simulink model "ModelLLCController"  (R2026a)
settings: Solver=ode23t  StopTime=5e-3  FixedStep=1e-4  MaxStep=1/(10*llcCompensator.resonantFrequency)  AbsTol=1e-3
PreLoadFcn:
  | % Parameterize the model
  | 
  | if ~exist('LLCDesign', 'var')
  | LLCConverterDefaultInputParameters;
  | end
undefined symbols (not defined in the file or in its folder): llcCompensator, LLCController
libraries: fl_lib x52, nesl_utility x34, ee_lib x27, ConverterLibrary x1
(part 1 of 4)
Description:
  | Design of LLC Resonant Converter
settings Model: SimulationMode=accelerator  ExtModeTrigDuration=100  Creator=The MathWorks, Inc.  LastModifiedBy=vsolaise
settings SolverCC: MaxConsecutiveMinStep=10
settings DataIOCC: StateSaveName=tmp_raccel_xout  SignalLoggingName=logsoutLLCConverter  OutputTimes=[0:1.1*3*Voc/(1*2000):1.1*3*Voc/1]
settings OptimizationCC: EfficientMapNaN2IntZero=off
settings HardwareCC: ProdHWDeviceType=Intel->x86-32 (Windows32)  TargetBitPerPointer=64.0  TargetBitPerSizeT=64.0  TargetBitPerPtrDiffT=64.0  TargetLongLongMode=on  TargetIntDivRoundTo=Zero  TargetEndianess=LittleEndian  TargetWordSize=64.0  TargetHWDeviceType=MATLAB Host  ProdEqTarget=off
settings RTWCC: SystemTargetFile=raccel.tlc  TemplateMakefile=raccel_default_tmf  RTWVerbose=off  RTWUseSimCustomCode=on
settings CodeAppCC: GenerateComments=off  MaxIdLength=128.0  SimulinkBlockComments=off
settings RaccelTargetCC: ExtModeTransport=0.0  ExtModeStaticAllocSize=1000000.0  ENABLE_SLEXEC_SSBRIDGE=1.0  RTWCAPIParams=on  RTWCAPIRootIO=on  MultiwordLength=2048.0
settings SimscapeCC: SimscapeNominalValues="[{\"value\":\"1\",\"unit\":\"A\"},{\"value\":\"1\",\"unit\":\"bar\"},{\"value\":\"1\",\"unit\":\"cm^2\"},{\"value\":\"1\",\"unit\":\"cm^3/s\"},{\"value\":\"1\",\"unit\":\"kJ/kg\"},{\"value\":\"1\",\"unit\":\"kW\"},{\"value\":\"1\",\"unit\":\"l\"},{\"value\":\"1\",\"unit\":\"N\"},{\"value\":\"1\",\"unit\":\"N*m\"},{\"value\":\"1\",\"unit\":\"V\"}]"  SimscapeLogName=SimlogLLCConverter  SimscapeLogLimitData=off  SimscapeLogDataHistory=5000.0

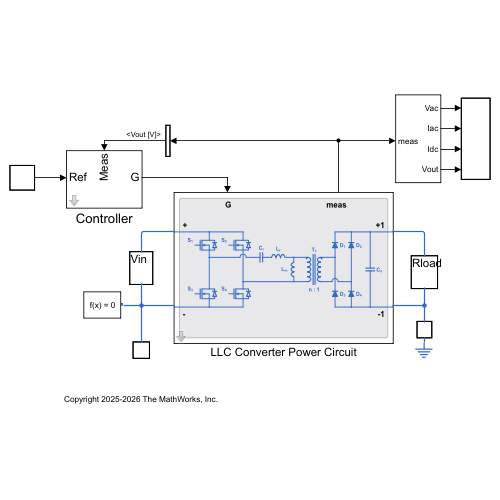
[thumbnail: Simulink's stored preview of the top-level diagram]
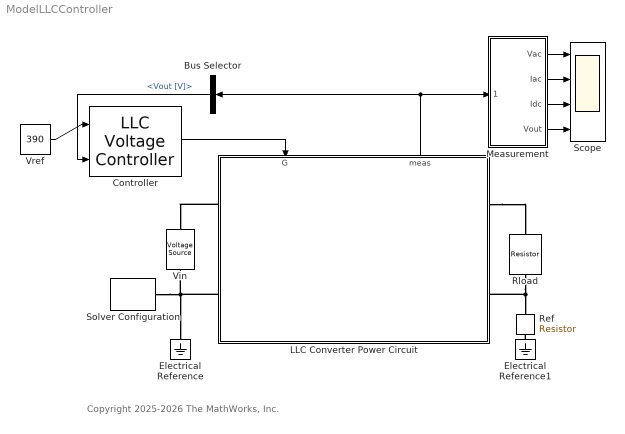
== system ModelLLCController ==
  note: Copyright 2025-2026 The MathWorks, Inc.
  Bus Selector : BusSelector  OutputSignals=Rectifier.Vout [V]
  Controller : ConverterLibrary/Controller/Soft-Switching Converters/LLC Voltage Controller  resFreq=llcCompensator.resonantFrequency  Fmin=llcCompensator.minPUfrequency  Fmax=llcCompensator.maxPUfrequency  Tdead=llcCompensator.deadTime  cntrlSelect=PI controller (Continuous)  VdcValue=LLCSpec.maxInputVoltage.value  Kc=llcCompensator.Ki  numSdomain=llcCompensator.numSDomain  denSdomain=llcCompensator.denSDomain  numZdomain=llcCompensator.numZDomain  denZdomain=llcCompensator.denZDomain  Kp=LLCController.Kp  Ki=LLCController.Ki  TsController=LLCController.Ts  vcoSelect=Two rate  vcoGain=llcCompensator.constantVCOGain  vcoGainVec=llcCompensator.constantVCOGain*[1 1]  pwmSampleTime=1e-7
      link override 2P2Z Compensator: LabelModeActiveChoice=PIContinuous
      link override VCO: LabelModeActiveChoice=TwoRate
      settings: SourceProductName=Simscape Power Converter Components
  Electrical Reference : fl_lib/Electrical/Electrical Elements/Electrical Reference
  Electrical Reference1 : fl_lib/Electrical/Electrical Elements/Electrical Reference
  LLC Converter Power Circuit : Subsystem  mask(LLC Converter Plant){llcConverterModel=Detailed Full-Bridge, ratedPower=10e3, ratedPower_unit=W, VIn=380, VIn_unit=V, Cr=3.3703e-7, Cr_unit=F, seriesInductorOption=Use transformer leakage inductance, Lr=30, Lr_unit=uH, RLr=0, RLr_unit=mOhm, Llk1=7.14e-6, Llk1_unit=H, R1=0.01, R1_unit=Ohm, Llk2=4.0645e-7, Llk2_unit=H, R2=0.01, R2_unit=Ohm, Lm=9.7705e-5, Lm_unit=H, n=0.96154, Cf=7.1111e-4, Cf_unit=F, Esr=0.02, Esr_unit=Ohm, Vco=350, Vco_unit=V, primaryDeviceOption=Ideal Semiconductor Switch, RdsOn=0.001, RdsOn_unit=Ohm, GdsOff=1e-5, GdsOff_unit=1/Ohm, Vth=2.5, Vth_unit=V, VfBody=0.6, VfBody_unit=V, RdBody=0.001, RdBody_unit=Ohm, GdBody=1e-5, GdBody_unit=1/Ohm, Cdsparasitic=2e-10, Cdsparasitic_unit=F, simTempPri=25, simTempPri_unit=degC, rectifierOption=Full Bridge, secondaryDeviceOption=Ideal Diode, VfSec=0.6, VfSec_unit=V, RdSec=0.001, RdSec_unit=Ohm, GdSec=1e-5, GdSec_unit=1/Ohm, simTempSec=25, simTempSec_unit=degC}
      mask prompts: llcConverterModel "LLC Converter model"; ratedPower "Rated power (P)"; VIn "Nominal input voltage (Vdc)"; Cr "Resonant capacitance (Cr)"; seriesInductorOption "Series resonant inductance"; Lr "Series resonant inductance (Lr)"; RLr "Series inductance resistance"; Llk1 "Primary leakage inductance (Lr)"; R1 "Primary resistance (R1)"; Llk2 "Secondary leakage inductance (Llk2)"; R2 "Secondary resistance (R2)"; Lm "Magnetizing inductance (Lm)"; n "Transformer turns ratio (n)"; Cf "Output filter capacitance (Co)"; Esr "Output filter capacitor ESR (Rco)"; Vco "Initial output capacitor voltage"; primaryDeviceOption "Select the primary switching device"; RdsOn "On-state resistance"; GdsOff "Off-state conductance"; Vth "Threshold voltage"; VfBody "Body diode forward voltage"; RdBody "Body diode on-resistance"; GdBody "Body diode off-conductance"; Cdsparasitic "MOSFET parasitic capacitance"; simTempPri "Simulation temperature"; rectifierOption "Select the rectifier topology"; secondaryDeviceOption "Select the secondary diode"; VfSec "Forward voltage"; RdSec "On resistance"; GdSec "Off conductance"; simTempSec "Simulation temperature"
      mask help: This block models the power circuit of the LLC resonant converter. You can choose between different switch and diode models. For the primary semiconductor switch, you can choose between ideal semiconductor switch, MOSFET without thermal port and tabulated MOSFET with thermal port. For the secondary, you can choose between ideal and tabulated diode.
      mask init:
      | %% Unit conversion: convert displayed values to base SI units
      | convMap = containers.Map( ...
      |     {'W','kW','MW','V','kV','mV','F','mF','uF','nF','pF', ...
      |      'H','mH','uH','nH','Ohm','kOhm','mOhm','S','mS','1/Ohm'}, ...
      |     {1, 1e3, 1e6, 1, 1e3, 1e-3, 1, 1e-3, 1e-6, 1e-9, 1e-12, ...
      |      1, 1e-3, 1e-6, 1e-9, 1, 1e3, 1e-3, 1, 1e-3, 1});
      | ratedPower = ratedPower * convMap(ratedPower_unit);
      | VIn = VIn * convMap(VIn_unit);
      | Cr = Cr * convMap(Cr_unit);
      | Lr_SI = Lr * convMap(Lr_unit);
      | RLr_SI = RLr * convMap(RLr_unit);
      | Llk1 = Llk1 * convMap(Llk1_unit);
      | R1 = R1 * convMap(R1_unit);
      | Llk2 = Llk2 * convMap(Llk2_unit);
      | R2 = R2 * convMap(R2_unit);
      | Lm = Lm * convMap(Lm_unit);
      | Cf = Cf * convMap(Cf_unit);
      | Esr = Esr * convMap(Esr_unit);
      | Vco_SI = Vco * convMap(Vco_unit);
      | RdsOn = RdsOn * convMap(RdsOn_unit);
      | GdsOff = GdsOff * convMap(GdsOff_unit);
      | Vth = Vth * convMap(Vth_unit);
      | VfBody = VfBody * convMap(VfBody_unit);
      | RdBody = RdBody * convMap(RdBody_unit);
      | GdBody = GdBody * convMap(GdBody_unit);
      | Cdsparasitic = Cdsparasitic * convMap(Cdsparasitic_unit);
      | VfSec = VfSec * convMap(VfSec_unit);
      | RdSec = RdSec * convMap(RdSec_unit);
      | GdSec = GdSec * convMap(GdSec_unit);
      | %% Transformer turns ratio and leakage inductances
      | % A centre-tap rectifier halves the ratio and doubles the secondary leakage of the
      | % centre-tapped transformer. With an external series inductor the leakages are a small
      | % share of it, referred to each winding, so they are never zero.
      | leakageShareOfExternalInductor = 1e-3;
      | primaryLeakage = Llk1;
      | secondaryLeakage = Llk2;
      | % Read by name: seriesInductorOption is an evaluated popup, so its workspace value is an index
      | if strcmp(get_param(gcb, 'seriesInductorOption'), 'Use external inductance') && startsWith(get_param(gcb, 'llcConverterModel'), 'Detailed')
      |     primaryLeakage = leakageShareOfExternalInductor*Lr_SI;
      |     secondaryLeakage = leakageShareOfExternalInductor*Lr_SI/n^2;
      | end
      | if ~(isfinite(primaryLeakage) && primaryLeakage > 0 && isfinite(secondaryLeakage) && secondaryLeakage > 0)
      |     error('The transformer leakage inductances must be positive. Primary: %g H, secondary: %g H.', ...
      |         primaryLeakage, secondaryLeakage);
      | end
      | if strcmp(rectifierOption, 'Centre-Tap')
      |     xfmrTurnsRatio = n/2;
      |     xfmrSecondaryLeakage = 2*secondaryLeakage;
      | else
      |     xfmrTurnsRatio = n;
      |     xfmrSecondaryLeakage = secondaryLeakage;
      | end
      | xfmrPrimaryLeakage = primaryLeakage;
      | %% Simulation temperature (loss-only, thermal MOSFET device)
      | % Temperature is an OFFSET unit (K = degC + 273.15), so it cannot use the
      | % multiplicative convMap above; convert it explicitly. simTempPri_K is read
      | % directly by each thermal MOSFET's junction-temperature initial target and by
      | % each Temperature Source in the primary bridge.
      | if strcmp(simTempPri_unit, 'degC')
      |     simTempPri_K = simTempPri + 273.15;
      | elseif strcmp(simTempPri_unit, 'K')
      |     simTempPri_K = simTempPri;
      | else
      |     error('LLC Converter Power Circuit: unrecognized simulation-temperature unit "%s" (expected degC or K).', simTempPri_unit);
      | end
      | %% Simulation temperature (secondary rectifier, tabulated diode)
      | % Same offset-unit conversion as the primary above (K = degC + 273.15), which is why
      | % neither can use the multiplicative convMap. simTempSec_K is read by every tabulated
      | % rectifier diode's device simulation temperature. That is the only temperature input
      | % those blocks have: in this configuration the diode has two electrical ports and no
      | % thermal port, so a junction-temperature target on it would be inert.
      | if strcmp(simTempSec_unit, 'degC')
      |     simTempSec_K = simTempSec + 273.15;
      | elseif strcmp(simTempSec_unit, 'K')
      |     simTempSec_K = simTempSec;
      | else
      |     error('LLC Converter Power Circuit: unrecognized simulation-temperature unit "%s" (expected degC or K).', simTempSec_unit);
      | end
      | %% Select model variant and visibility
      | selectLLCPlantModel(gcb);
      | %% Block icon
      | % The icon is drawn by the mask Display code, which resolves its four artwork files
      | % (FullBridgeLLCCentreTapRectifier.svg and siblings) by name from the MATLAB path.
      | % They live in Components/ConverterPlants/CombinedLLCConverterPlant/icons, which
      | % the project puts on the path. An earlier design kept the SVG source in
      | % model-workspace variables and unpacked it to tempdir here; those variables no longer
      | % exist, so that code only stranded a file handle on a zero-byte temp file every run.
      settings: CopyFcn="set_param(gcbh,\"LinkStatus\",\"none\");"  PortSchema="{\"entries\":[{\"content\":{\"sides\":[{\"content\":{\"connectorIds\":[\"LConn1\",\"LConn2\"]},\"type\":\"ConnectorPlacement.EquallySpacedRectSide\",\"uuid\":\"7d0af355-cbc1-43de-86a8-478c0417a0e6\"},{\"content\":{\"connectorIds\":[\"RConn1\",\"RConn2\"],\"side\":\"RIGHT\"},\"type\":\"ConnectorPlacement.EquallySpacedRectSide\",\"uuid\":\"e5e2e9fd-b3a0-4f29-84de-d1d266c8101b\"},{\"content\":{\"connectorIds\":[\"In1\",\"Out1\"],\"side\":\"TOP\"},\"type\":\"ConnectorPlacement.EquallySpacedRectSide\",\"uuid\":\"2a0404a0-819d-4dd0-9f33-52ca4a6707b9\"}]},\"type\":\"ConnectorPlacement.EquallySpacedConnector\",\"uuid\":\"862cc0c4-78b7-4235-be37-b455f1ccafcc\"}],\"packageUris\":[\"http://schema.mathworks.com/mf0/Connector/R2020b\"],\"version\":\"1.0\"}"
      mask Help: web('LLCConverterPlant.html')
      mask TypeOptions llcConverterModel: Simplified Half-Bridge | Detailed Half-Bridge | Detailed Full-Bridge
      mask Callback llcConverterModel: selectLLCPlantModel(gcb);
      mask TypeOptions ratedPower_unit: W | kW | MW
      mask TypeOptions VIn_unit: V | kV | mV
      mask TypeOptions Cr_unit: F | mF | uF | nF | pF
      mask TypeOptions seriesInductorOption: Use external inductance | Use transformer leakage inductance
      mask Callback seriesInductorOption: selectLLCSeriesInductor(gcb);
      mask TypeOptions Lr_unit: H | mH | uH | nH
      mask TypeOptions RLr_unit: Ohm | mOhm | kOhm
      mask TypeOptions Llk1_unit: H | mH | uH | nH
      mask TypeOptions R1_unit: Ohm | kOhm | mOhm
      mask TypeOptions Llk2_unit: H | mH | uH | nH
      mask TypeOptions R2_unit: Ohm | kOhm | mOhm
      mask TypeOptions Lm_unit: H | mH | uH | nH
      mask TypeOptions Cf_unit: F | mF | uF | nF | pF
      mask TypeOptions Esr_unit: Ohm | kOhm | mOhm
      mask TypeOptions Vco_unit: V | kV | mV
      mask TypeOptions primaryDeviceOption: Ideal Semiconductor Switch | MOSFET (Ideal, Switching) with Thermal
      mask Callback primaryDeviceOption: selectLLCPlantPrimaryMOSFET(gcb);
      mask TypeOptions RdsOn_unit: Ohm | kOhm | mOhm
      mask TypeOptions GdsOff_unit: 1/Ohm | S | mS
      mask TypeOptions Vth_unit: V | kV | mV
      mask TypeOptions VfBody_unit: V | mV
      mask TypeOptions RdBody_unit: Ohm | kOhm | mOhm
      mask TypeOptions GdBody_unit: 1/Ohm | S | mS
      mask TypeOptions Cdsparasitic_unit: F | mF | uF | nF | pF
      mask TypeOptions simTempPri_unit: degC | K
      mask TypeOptions rectifierOption: Centre-Tap | Full Bridge
      mask Callback rectifierOption: selectLLCPlantSecondaryDiode(gcb);
      mask TypeOptions secondaryDeviceOption: Ideal Diode | Tabulated Diode
      mask Callback secondaryDeviceOption: selectLLCPlantSecondaryDiode(gcb);
      mask TypeOptions VfSec_unit: V | mV
      mask TypeOptions RdSec_unit: Ohm | kOhm | mOhm
      mask TypeOptions GdSec_unit: 1/Ohm | S | mS
      mask TypeOptions simTempSec_unit: degC | K
      mask DialogControl LLCTank Prompt: Resonant tank parameters
      mask DialogControl Switch Prompt: Primary Inverter
      mask DialogControl openMOSFETMask Prompt: Open the MOSFET block mask
      mask DialogControl openMOSFETMask Callback:
      | blockPath = [gcb, '/LLC Primary Inverter and Resonant Tank/LLC Detailed Model/Inverter/Primary Inverter'];
      | llcConverterChoice = get_param(gcb,'llcConverterModel');
      | switch llcConverterChoice
      |     case 'Detailed Half-Bridge'
      |         open_system([blockPath, '/Half Bridge with Thermal/MOSFETA1'], 'mask');
      |     case 'Detailed Full-Bridge'
      |         open_system([blockPath, '/Full Bridge with Thermal/MOSFETA1'], 'mask');
      |     otherwise
      |         error('Open the MOSFET mask only in a Detailed model with the thermal MOSFET device selected.');
      | end
      mask DialogControl applyMOSFETParam Prompt: Apply parameters to all primary MOSFET blocks
      mask DialogControl applyMOSFETParam Callback:
      | llcConverterChoice = get_param(gcb, 'llcConverterModel');
      | primaryInvBase = [gcb, '/LLC Primary Inverter and Resonant Tank/LLC Detailed Model/Inverter/Primary Inverter'];
      | switch llcConverterChoice
      |     case 'Detailed Half-Bridge'
      |         srcBlock = [primaryInvBase, '/Half Bridge with Thermal/MOSFETA1'];
      |         dstBlocks = {[primaryInvBase, '/Half Bridge with Thermal/MOSFETA2']};
      |     case 'Detailed Full-Bridge'
      |         srcBlock = [primaryInvBase, '/Full Bridge with Thermal/MOSFETA1'];
      |         dstBlocks = {[primaryInvBase, '/Full Bridge with Thermal/MOSFETA2'], [primaryInvBase, '/Full Bridge with Thermal/MOSFETB1'], [primaryInvBase, '/Full Bridge with Thermal/MOSFETB2']};
      |     otherwise
      |         return;
      | end
      | paramNames = fieldnames(get_param(srcBlock, 'DialogParameters'));
      | paramValues = cellfun(@(x) get_param(srcBlock, x), paramNames, 'UniformOutput', false);
      | for k = 1:numel(dstBlocks)
      |     cellfun(@(x, y) set_param(dstBlocks{k}, x, y), paramNames, paramValues, 'UniformOutput', false);
      | end
      | fprintf('Applied MOSFET parameters to %d blocks.\n', numel(dstBlocks));
      mask DialogControl Diode Prompt: Secondary Rectifier
      mask DialogControl openDiodeMask Prompt: Open the Diode block mask
      mask DialogControl openDiodeMask Callback:
      | rectBridge = [gcb, '/Rectifier/Rectifier Bridge'];
      | if strcmp(get_param(gcb, 'rectifierOption'), 'Centre-Tap')
      |     diodeBlk = [rectBridge, '/Centre-Tap Tabulated Diode/Diode1'];
      | else
      |     diodeBlk = [rectBridge, '/Full Bridge Tabulated Diode/Diode1'];
      | end
      | open_system(diodeBlk, 'mask');
      mask DialogControl applyDiodeParam Prompt: Apply parameters to all secondary Diode blocks
      mask DialogControl applyDiodeParam Callback:
      | rectBridge = [gcb, '/Rectifier/Rectifier Bridge'];
      | if strcmp(get_param(gcb, 'rectifierOption'), 'Centre-Tap')
      |     subsys = [rectBridge, '/Centre-Tap Tabulated Diode'];
      | else
      |     subsys = [rectBridge, '/Full Bridge Tabulated Diode'];
      | end
      | srcBlock = [subsys, '/Diode1'];
      | dstBlocks = find_system(subsys, 'SearchDepth', 1, 'LookUnderMasks', 'all', 'BlockType', 'SimscapeBlock');
      | dstBlocks(strcmp(dstBlocks, srcBlock)) = [];
      | dstBlocks(contains(dstBlocks, 'Open Circuit')) = [];
      | paramNames = fieldnames(get_param(srcBlock, 'DialogParameters'));
      | paramValues = cellfun(@(x) get_param(srcBlock, x), paramNames, 'UniformOutput', false);
      | for k = 1:numel(dstBlocks)
      |     cellfun(@(x, y) set_param(dstBlocks{k}, x, y), paramNames, paramValues, 'UniformOutput', false);
      | end
      | fprintf('Applied Diode1 parameters to %d other diode blocks.\\n', numel(dstBlocks));
      mask DialogControl ExportPanel Prompt: Export to Unmasked Subsystem
      mask DialogControl ExportInfo Prompt: To customize the converter, export it as an unmasked subsystem with the active variant flattened - a standalone, fully-editable circuit plus a parameter file. Requires the "Variant Manager for Simulink" add-on.
      mask DialogControl exportToModel Prompt: Export
      mask DialogControl exportToModel Callback: exportConverterModelFromMask(gcb);
      mask Display:
      | llcModel = get_param(gcb, 'llcConverterModel');
      | rectOpt = get_param(gcb, 'rectifierOption');
      | if strcmp(llcModel, 'Detailed Full-Bridge')
      |     if strcmp(rectOpt, 'Full Bridge')
      |         image('FullBridgeLLCFullBridgeRectifier.svg', [0 0 1 1]);
      |     else
      |         image('FullBridgeLLCCentreTapRectifier.svg', [0 0 1 1]);
      |     end
      | else
      |     if strcmp(rectOpt, 'Full Bridge')
      |         image('HalfBridgeLLCFullBridgeRectifier.svg', [0 0 1 1]);
      |     else
      |         image('HalfBridgeLLCCentreTapRectifier.svg', [0 0 1 1]);
      |     end
      | end
  Measurement : Subsystem
  Ref : fl_lib/Electrical/Electrical Elements/Resistor  R=1e5 Ohm  i_specify=off  i_priority=None  i=0 A  i_nominal_specify=off  i_nominal_value=1  i_nominal_unit=A  v_specify=off  v_priority=None  v=0 V  v_nominal_specify=off  v_nominal_value=1  v_nominal_unit=V
  Rload : fl_lib/Electrical/Electrical Elements/Resistor  R=20.48 Ohm  i_specify=off  i_priority=None  i=0 A  i_nominal_specify=off  i_nominal_value=1  i_nominal_unit=A  v_specify=off  v_priority=None  v=0 V  v_nominal_specify=off  v_nominal_value=1  v_nominal_unit=V
  Scope : Scope  NumInputPorts=4
      settings: Title=Resonant Tank Voltages  ActiveDisplayYMinimum=-493.54853502129527  ActiveDisplayYMaximum=493.54967336166339
  Solver Configuration : nesl_utility/Solver Configuration  PhysicalDomain=network_engine_domain  SubClassName=solver  LeftPortType=input  RightPortType=generic  Tones=[]  Harmonics=[]  SimulateNoise=off  Profile=off  UseLocalSampling=off  EnableSwitchedLinearOptims=on  FrequencyDomain=off  UseCCode=off  RelTol=0.001  AbsTol=0.001  MinStep=1e-09  ToWorkspace=off  RevertToSquareIcSolve=off  NumHomotopyIterations=100  PhasorMode=off  PhasorModeNumHarmonics=1  ConsistencySolver=NEWTON_XTOL_AFTER_FTOL  CanonicalOrdering=UNORDERED  OptimizeIntermediates=UNOPTIMIZED  IndexReductionMethod=DerivativeReplacement  DoDC=off  ResidualTolerance=1e-09  ConsistencyTolSource=GLOBAL  ConsistencyAbsTol=0.001  ConsistencyRelTol=0.001  ConsistencyTolFactor=0.001  UseLocalSolver=on  LocalSolverChoice=NE_BACKWARD_EULER_ADVANCER  ResolveIndetEquations=off  FunctionEvalNumThread=1  LocalSolverSampleTime=1e-7  DoFixedCost=on  MaxNonlinIter=3  MaxModeIter=10  ComputeImpulses=off  ImpulseIterations=2  LinearAlgebra=auto  LinearAlgebraNumThread=0  EquationFormulation=NE_TIME_EF  DelaysMemoryBudget=1024  AutomaticFiltering=on  FilteringTimeConstant=0.001  PartitionStorageMethod=AS_NEEDED  PartitionMemoryBudget=1024  PartitionMethod=ROBUST  MultibodyUseLocalSolver=off  MultibodyLocalSolverChoice=ODE1  MultibodyLocalSolverSampleTime=0.001
  Vin : ee_lib/Sources/Voltage Source  dc_voltage=385 V  ac_voltage=0 V  ac_shift=0 rad  ac_frequency=0 Hz  noise_mode=ee.enum.sources.noise.Disabled  PSD=0 V^2/Hz  sample_time=1e-3 s  repeatability=ee.enum.sources.repeatability.NotRepeatable  user_seed=0  auto_seed=3499211588  i_specify=off  i_priority=None  i=0 A  i_nominal_specify=off  i_nominal_value=1  i_nominal_unit=A  v_specify=off  v_priority=None  v=0 V  v_nominal_specify=off  v_nominal_value=1  v_nominal_unit=V
  Vref : Constant  Value=390
  wires:
  Measurement/1(Vac) -> Scope/1
  Measurement/2(Iac) -> Scope/2
  Measurement/3(Idc) -> Scope/3
  Measurement/4(Vout) -> Scope/4
  Bus Selector/1 -> Controller/2  "<Vout [V]>"
  Vref/1 -> Controller/1
  Controller/1 -> LLC Converter Power Circuit/1(G)
  LLC Converter Power Circuit/1(meas) -> Bus Selector/1, Measurement/1(meas)
  connections:
  Electrical Reference1/LConn1 -- Ref/RConn1
  Rload/RConn1 -- Ref/LConn1 -- LLC Converter Power Circuit/RConn2
  LLC Converter Power Circuit/LConn1 -- Vin/LConn1
  LLC Converter Power Circuit/RConn1 -- Rload/LConn1
  Solver Configuration/RConn1 -- Electrical Reference/LConn1 -- LLC Converter Power Circuit/LConn2 -- Vin/RConn1

== system ModelLLCController/LLC Converter Power Circuit ==
  G : Inport
  Bus Creator : BusCreator  Inputs=3
  LLC Primary Inverter and Resonant Tank : Subsystem  Variant=on  VariantControlMode=label  LabelModeActiveChoice=DetailedModel
  Rectifier : Subsystem
      settings: PortSchema="{\"entries\":[{\"content\":{\"sides\":[{\"content\":{\"connectorIds\":[\"LConn1\",\"LConn2\",\"LConn3\"]},\"type\":\"ConnectorPlacement.EquallySpacedRectSide\",\"uuid\":\"4786b3cc-2245-4c72-a50b-9c63e4ad3d8a\"},{\"content\":{\"connectorIds\":[\"RConn1\",\"RConn2\"],\"side\":\"RIGHT\"},\"type\":\"ConnectorPlacement.EquallySpacedRectSide\",\"uuid\":\"250a01d0-bf95-4e01-bf69-d866bcf3b7bd\"},{\"content\":{\"connectorIds\":[\"Out1\"],\"side\":\"TOP\"},\"type\":\"ConnectorPlacement.EquallySpacedRectSide\",\"uuid\":\"52730d18-084b-4644-8b2a-b54c84fa88ec\"}]},\"type\":\"ConnectorPlacement.EquallySpacedConnector\",\"uuid\":\"d24cae2a-f132-4f5a-ac35-d7440d7a99e9\"}],\"packageUris\":[\"http://schema.mathworks.com/mf0/Connector/R2020b\"],\"version\":\"1.0\"}"
  + : PMIOPort  Side=Left
  +1 : PMIOPort  Port=2  Side=Right
  - : PMIOPort  Port=3  Side=Left
  -1 : PMIOPort  Port=4  Side=Right
  meas : Outport
  wires:
  Rectifier/1(meas) -> Bus Creator/3  "Rectifier"
  G/1 -> LLC Primary Inverter and Resonant Tank/1(G)
  LLC Primary Inverter and Resonant Tank/1(measInv) -> Bus Creator/1
  LLC Primary Inverter and Resonant Tank/2(measTank) -> Bus Creator/2
  Bus Creator/1 -> meas/1
  connections:
  +1/RConn1 -- Rectifier/RConn1
  -1/RConn1 -- Rectifier/RConn2
  LLC Primary Inverter and Resonant Tank/LConn1 -- +/RConn1
  LLC Primary Inverter and Resonant Tank/LConn2 -- -/RConn1
  LLC Primary Inverter and Resonant Tank/RConn1 -- Rectifier/LConn1
  LLC Primary Inverter and Resonant Tank/RConn2 -- Rectifier/LConn2
  LLC Primary Inverter and Resonant Tank/RConn3 -- Rectifier/LConn3

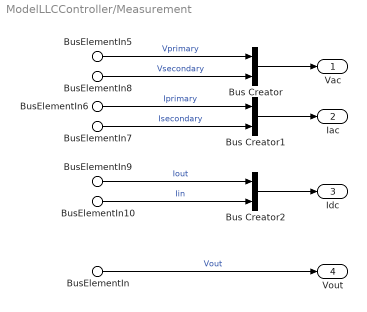
== system ModelLLCController/Measurement ==
  BusElementIn7 : Inport  PortName=meas  Element=Rectifier.Is [A]
  BusElementIn9 : Inport  PortName=meas  Element=Rectifier.Iout [A]
  BusElementIn : Inport  PortName=meas  Element=Rectifier.Vout [V]
  BusElementIn10 : Inport  PortName=meas  Element=Inverter.Iin [A]
  BusElementIn5 : Inport  PortName=meas  Element=ResonantTank.Vp [V]
  BusElementIn6 : Inport  PortName=meas  Element=ResonantTank.Ip [A]
  BusElementIn8 : Inport  PortName=meas  Element=ResonantTank.Vs [A]
  Bus Creator : BusCreator  Inputs=2
  Bus Creator1 : BusCreator  Inputs=2
  Bus Creator2 : BusCreator  Inputs=2
  Vac : Outport
  Iac : Outport  Port=2
  Idc : Outport  Port=3
  Vout : Outport  Port=4
  wires:
  BusElementIn5/1 -> Bus Creator/1  "Vprimary"
  BusElementIn8/1 -> Bus Creator/2  "Vsecondary"
  BusElementIn6/1 -> Bus Creator1/1  "Iprimary"
  BusElementIn7/1 -> Bus Creator1/2  "Isecondary"
  Bus Creator1/1 -> Iac/1
  BusElementIn10/1 -> Bus Creator2/2  "Iin"
  Bus Creator2/1 -> Idc/1
  BusElementIn9/1 -> Bus Creator2/1  "Iout"
  BusElementIn/1 -> Vout/1  "Vout"
  Bus Creator/1 -> Vac/1

== system ModelLLCController/LLC Converter Power Circuit/LLC Primary Inverter and Resonant Tank ==
  G : Inport
  LLC Detailed Model : Subsystem  VariantControl=DetailedModel
  LLC Simplified Model : Subsystem  VariantControl=SimplifiedModel
  + : PMIOPort  Side=Left
  - : PMIOPort  Port=2  Side=Left
  P2+ : PMIOPort  Port=3  Side=Right
  N2 : PMIOPort  Port=4  Side=Right
  P2- : PMIOPort  Port=5  Side=Right
  measInv : Outport
  measTank : Outport  Port=2

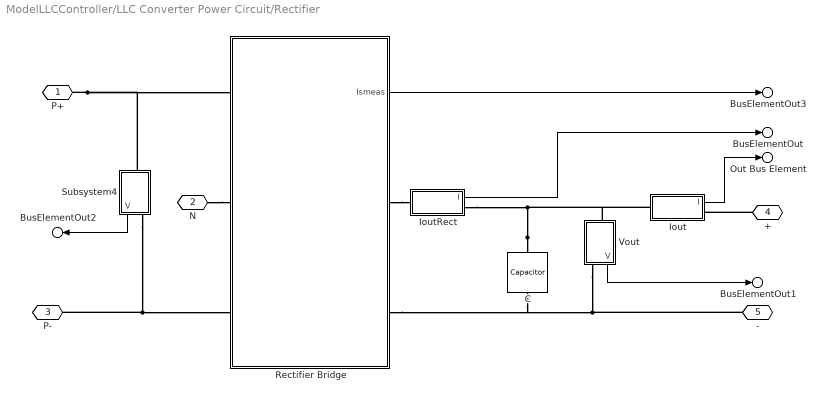
== system ModelLLCController/LLC Converter Power Circuit/Rectifier ==
  C : fl_lib/Electrical/Electrical Elements/Capacitor  c=Cf F  r=Esr Ohm  g=0 1/Ohm  i_specify=off  i_priority=None  i=0 A  i_nominal_specify=off  i_nominal_value=1  i_nominal_unit=A  v_specify=off  v_priority=None  v=450 V  v_nominal_specify=off  v_nominal_value=1  v_nominal_unit=V  vc_specify=on  vc_priority=High  vc=Vco_SI V  vc_nominal_specify=off  vc_nominal_value=1  vc_nominal_unit=V
  Iout : Subsystem
      mask Display: disp("I")
  IoutRect : Subsystem
      mask Display: disp("I")
  Rectifier Bridge : Subsystem  Variant=on  VariantControlMode=label  LabelModeActiveChoice=FullBridgeIdealDiode
  Subsystem4 : Subsystem
      settings: PortSchema="{\"entries\":[{\"content\":{\"sides\":[{\"content\":{\"connectorIds\":[\"LConn1\"]},\"type\":\"ConnectorPlacement.EquallySpacedRectSide\",\"uuid\":\"e749c2ff-fd60-426f-a769-b61a7dfe80d2\"},{\"content\":{\"connectorIds\":[\"RConn1\",\"Out1\"],\"side\":\"RIGHT\"},\"type\":\"ConnectorPlacement.EquallySpacedRectSide\",\"uuid\":\"f3bb02bd-f8d2-4326-b68c-6f969fa4ac22\"},{\"content\":{\"side\":\"TOP\"},\"type\":\"ConnectorPlacement.EquallySpacedRectSide\",\"uuid\":\"9ab7a0d1-20d8-49e4-8eb3-54d34434204c\"}]},\"type\":\"ConnectorPlacement.EquallySpacedConnector\",\"uuid\":\"19e2a6d5-13f4-47de-bb59-b826817cba83\"}],\"packageUris\":[\"http://schema.mathworks.com/mf0/Connector/R2020b\"],\"version\":\"1.0\"}"
      mask Display: disp("V")
  Vout : Subsystem
      settings: PortSchema="{\"entries\":[{\"content\":{\"sides\":[{\"content\":{\"connectorIds\":[\"LConn1\"]},\"type\":\"ConnectorPlacement.EquallySpacedRectSide\",\"uuid\":\"e749c2ff-fd60-426f-a769-b61a7dfe80d2\"},{\"content\":{\"connectorIds\":[\"RConn1\",\"Out1\"],\"side\":\"RIGHT\"},\"type\":\"ConnectorPlacement.EquallySpacedRectSide\",\"uuid\":\"f3bb02bd-f8d2-4326-b68c-6f969fa4ac22\"},{\"content\":{\"side\":\"TOP\"},\"type\":\"ConnectorPlacement.EquallySpacedRectSide\",\"uuid\":\"9ab7a0d1-20d8-49e4-8eb3-54d34434204c\"}]},\"type\":\"ConnectorPlacement.EquallySpacedConnector\",\"uuid\":\"19e2a6d5-13f4-47de-bb59-b826817cba83\"}],\"packageUris\":[\"http://schema.mathworks.com/mf0/Connector/R2020b\"],\"version\":\"1.0\"}"
      mask Display: disp("V")
  P+ : PMIOPort  Side=Left
  N : PMIOPort  Port=2  Side=Left
  P- : PMIOPort  Port=3  Side=Left
  + : PMIOPort  Port=4  Side=Right
  - : PMIOPort  Port=5  Side=Right
  Out Bus Element : Outport  PortName=meas  Element=Iout [A]
  BusElementOut : Outport  PortName=meas  Element=IL [A]
  BusElementOut1 : Outport  PortName=meas  Element=Vout [V]
  BusElementOut2 : Outport  PortName=meas  Element=Vac [V]
  BusElementOut3 : Outport  PortName=meas  Element=Is [A]
  wires:
  Rectifier Bridge/1(Ismeas) -> BusElementOut3/1
  Subsystem4/1(V) -> BusElementOut2/1
  Vout/1(V) -> BusElementOut1/1
  IoutRect/1(I) -> BusElementOut/1
  Iout/1(I) -> Out Bus Element/1
  connections:
  +/RConn1 -- Iout/RConn1
  C/LConn1 -- IoutRect/RConn1 -- Iout/LConn1 -- Vout/LConn1
  -/RConn1 -- Rectifier Bridge/RConn2 -- C/RConn1 -- Vout/RConn1
  P+/RConn1 -- Subsystem4/LConn1 -- Rectifier Bridge/LConn1
  Subsystem4/RConn1 -- Rectifier Bridge/LConn3 -- P-/RConn1
  N/RConn1 -- Rectifier Bridge/LConn2
  Rectifier Bridge/RConn1 -- IoutRect/LConn1

== system ModelLLCController/LLC Converter Power Circuit/LLC Primary Inverter and Resonant Tank/LLC Detailed Model ==
  G : Inport
  Inverter : Subsystem
      settings: PortSchema="{\"entries\":[{\"content\":{\"sides\":[{\"content\":{\"connectorIds\":[\"LConn1\",\"LConn2\"]},\"type\":\"ConnectorPlacement.EquallySpacedRectSide\",\"uuid\":\"5f98eff0-54e4-47a8-aeeb-0279cba14f26\"},{\"content\":{\"connectorIds\":[\"RConn1\",\"RConn2\"],\"side\":\"RIGHT\"},\"type\":\"ConnectorPlacement.EquallySpacedRectSide\",\"uuid\":\"71acbbb6-1fc8-426c-b389-5d494eb18bfd\"},{\"content\":{\"connectorIds\":[\"In1\",\"Out1\"],\"side\":\"TOP\"},\"type\":\"ConnectorPlacement.EquallySpacedRectSide\",\"uuid\":\"dc77ee05-1f57-4323-bfda-b0076e2d1ee5\"}]},\"type\":\"ConnectorPlacement.EquallySpacedConnector\",\"uuid\":\"8d0b8c05-d5c5-4033-af60-ebdb639bdc40\"}],\"packageUris\":[\"http://schema.mathworks.com/mf0/Connector/R2020b\"],\"version\":\"1.0\"}"
  Resonant Tank : Subsystem
      settings: PortSchema="{\"entries\":[{\"content\":{\"sides\":[{\"content\":{\"connectorIds\":[\"LConn1\",\"LConn2\"]},\"type\":\"ConnectorPlacement.EquallySpacedRectSide\",\"uuid\":\"d505f362-3b8e-4dee-9b5b-731d75550efb\"},{\"content\":{\"connectorIds\":[\"RConn1\",\"RConn2\",\"RConn3\"],\"side\":\"RIGHT\"},\"type\":\"ConnectorPlacement.EquallySpacedRectSide\",\"uuid\":\"66ab4b84-9b7a-404b-b3f6-3ac1c371ea42\"},{\"content\":{\"connectorIds\":[\"Out1\"],\"side\":\"TOP\"},\"type\":\"ConnectorPlacement.EquallySpacedRectSide\",\"uuid\":\"00605859-d490-4a3b-aace-391362dfba7e\"}]},\"type\":\"ConnectorPlacement.EquallySpacedConnector\",\"uuid\":\"a210fe68-7181-499f-8e1c-ccfe71b42a4c\"}],\"packageUris\":[\"http://schema.mathworks.com/mf0/Connector/R2020b\"],\"version\":\"1.0\"}"
      mask Display: image('LLCTransformerIcon.png');
  + : PMIOPort  Side=Left
  P2+ : PMIOPort  Port=2  Side=Right
  N2 : PMIOPort  Port=3  Side=Right
  - : PMIOPort  Port=4  Side=Left
  P2- : PMIOPort  Port=5  Side=Right
  measInv : Outport
  measTank : Outport  Port=2
  wires:
  G/1 -> Inverter/1(G)
  Inverter/1(meas) -> measInv/1  "Inverter"
  Resonant Tank/1(meas) -> measTank/1  "ResonantTank"
  connections:
  -/RConn1 -- Inverter/LConn2
  Resonant Tank/LConn1 -- Inverter/RConn1
  Resonant Tank/RConn3 -- P2-/RConn1
  Resonant Tank/LConn2 -- Inverter/RConn2
  Resonant Tank/RConn1 -- P2+/RConn1
  +/RConn1 -- Inverter/LConn1
  Resonant Tank/RConn2 -- N2/RConn1

== system ModelLLCController/LLC Converter Power Circuit/LLC Primary Inverter and Resonant Tank/LLC Simplified Model ==
  G : Inport
  Inverter : Subsystem
      settings: PortSchema="{\"entries\":[{\"content\":{\"sides\":[{\"content\":{\"connectorIds\":[\"LConn1\",\"LConn2\"]},\"type\":\"ConnectorPlacement.EquallySpacedRectSide\",\"uuid\":\"5f98eff0-54e4-47a8-aeeb-0279cba14f26\"},{\"content\":{\"connectorIds\":[\"RConn1\",\"RConn2\"],\"side\":\"RIGHT\"},\"type\":\"ConnectorPlacement.EquallySpacedRectSide\",\"uuid\":\"71acbbb6-1fc8-426c-b389-5d494eb18bfd\"},{\"content\":{\"connectorIds\":[\"In1\",\"Out1\"],\"side\":\"TOP\"},\"type\":\"ConnectorPlacement.EquallySpacedRectSide\",\"uuid\":\"dc77ee05-1f57-4323-bfda-b0076e2d1ee5\"}]},\"type\":\"ConnectorPlacement.EquallySpacedConnector\",\"uuid\":\"8d0b8c05-d5c5-4033-af60-ebdb639bdc40\"}],\"packageUris\":[\"http://schema.mathworks.com/mf0/Connector/R2020b\"],\"version\":\"1.0\"}"
  Resonant Tank : Subsystem
      settings: PortSchema="{\"entries\":[{\"content\":{\"sides\":[{\"content\":{\"connectorIds\":[\"LConn1\",\"LConn2\"]},\"type\":\"ConnectorPlacement.EquallySpacedRectSide\",\"uuid\":\"d505f362-3b8e-4dee-9b5b-731d75550efb\"},{\"content\":{\"connectorIds\":[\"RConn1\",\"RConn2\",\"RConn3\"],\"side\":\"RIGHT\"},\"type\":\"ConnectorPlacement.EquallySpacedRectSide\",\"uuid\":\"66ab4b84-9b7a-404b-b3f6-3ac1c371ea42\"},{\"content\":{\"connectorIds\":[\"Out1\"],\"side\":\"TOP\"},\"type\":\"ConnectorPlacement.EquallySpacedRectSide\",\"uuid\":\"00605859-d490-4a3b-aace-391362dfba7e\"}]},\"type\":\"ConnectorPlacement.EquallySpacedConnector\",\"uuid\":\"a210fe68-7181-499f-8e1c-ccfe71b42a4c\"}],\"packageUris\":[\"http://schema.mathworks.com/mf0/Connector/R2020b\"],\"version\":\"1.0\"}"
      mask Display: image('LLCTransformerIcon.png');
  Selector : Selector  InputPortWidth=4  IndexOptions=Index vector (dialog)  Indices=[1 2]  OutputSizes=1
  + : PMIOPort  Side=Left
  P2+ : PMIOPort  Port=2  Side=Right
  N2 : PMIOPort  Port=3  Side=Right
  - : PMIOPort  Port=4  Side=Left
  P2- : PMIOPort  Port=5  Side=Right
  measInv : Outport
  measTank : Outport  Port=2
  wires:
  Inverter/1(meas) -> measInv/1  "Inverter"
  Resonant Tank/1(meas) -> measTank/1  "ResonantTank"
  G/1 -> Selector/1
  Selector/1 -> Inverter/1(G)
  connections:
  -/RConn1 -- Inverter/LConn2
  Resonant Tank/LConn1 -- Inverter/RConn1
  Resonant Tank/RConn3 -- P2-/RConn1
  Resonant Tank/LConn2 -- Inverter/RConn2
  Resonant Tank/RConn1 -- P2+/RConn1
  +/RConn1 -- Inverter/LConn1
  Resonant Tank/RConn2 -- N2/RConn1

== system ModelLLCController/LLC Converter Power Circuit/Rectifier/Iout ==
  Current Sensor : fl_lib/Electrical/Electrical Sensors/Current Sensor
  PS-Simulink Converter : nesl_utility/PS-Simulink Converter  PhysicalDomain=network_engine_domain  SubClassName=ps_output  LeftPortType=input  RightPortType=output  PseudoPeriodic=off  Frequencies=[]  VectorFormat=inherit  Unit=inherit  AffineConversion=off
  + : PMIOPort  Side=Left
  - : PMIOPort  Port=2  Side=Right
  I : Outport
  wires:
  PS-Simulink Converter/1 -> I/1
  connections:
  Current Sensor/RConn2 -- -/RConn1
  +/RConn1 -- Current Sensor/LConn1
  Current Sensor/RConn1 -- PS-Simulink Converter/LConn1

== system ModelLLCController/LLC Converter Power Circuit/Rectifier/IoutRect ==
  Current Sensor : fl_lib/Electrical/Electrical Sensors/Current Sensor
  PS-Simulink Converter : nesl_utility/PS-Simulink Converter  PhysicalDomain=network_engine_domain  SubClassName=ps_output  LeftPortType=input  RightPortType=output  PseudoPeriodic=off  Frequencies=[]  VectorFormat=inherit  Unit=inherit  AffineConversion=off
  + : PMIOPort  Side=Left
  - : PMIOPort  Port=2  Side=Right
  I : Outport
  wires:
  PS-Simulink Converter/1 -> I/1
  connections:
  Current Sensor/RConn2 -- -/RConn1
  +/RConn1 -- Current Sensor/LConn1
  Current Sensor/RConn1 -- PS-Simulink Converter/LConn1

== system ModelLLCController/LLC Converter Power Circuit/Rectifier/Rectifier Bridge ==
  Centre-Tap Ideal Diode : Subsystem  VariantControl=CentreTapIdealDiode
  Centre-Tap Tabulated Diode : Subsystem  VariantControl=CentreTapTabulatedDiode
  Full Bridge Ideal Diode : Subsystem  VariantControl=FullBridgeIdealDiode
  Full Bridge Tabulated Diode : Subsystem  VariantControl=FullBridgeTabulatedDiode
  P1+ : PMIOPort  Side=Left
  N1 : PMIOPort  Port=2  Side=Left
  P1- : PMIOPort  Port=3  Side=Left
  P2 : PMIOPort  Port=4  Side=Right
  N2 : PMIOPort  Port=5  Side=Right
  Ismeas : Outport

== system ModelLLCController/LLC Converter Power Circuit/Rectifier/Subsystem4 ==
  PS-Simulink Converter : nesl_utility/PS-Simulink Converter  PhysicalDomain=network_engine_domain  SubClassName=ps_output  LeftPortType=input  RightPortType=output  PseudoPeriodic=off  Frequencies=[]  VectorFormat=inherit  Unit=inherit  AffineConversion=off
  Voltage Sensor : fl_lib/Electrical/Electrical Sensors/Voltage Sensor
  + : PMIOPort  Side=Left
  - : PMIOPort  Port=2  Side=Right
  V : Outport
  wires:
  PS-Simulink Converter/1 -> V/1
  connections:
  Voltage Sensor/RConn2 -- -/RConn1
  Voltage Sensor/LConn1 -- +/RConn1
  PS-Simulink Converter/LConn1 -- Voltage Sensor/RConn1

== system ModelLLCController/LLC Converter Power Circuit/Rectifier/Vout ==
  PS-Simulink Converter : nesl_utility/PS-Simulink Converter  PhysicalDomain=network_engine_domain  SubClassName=ps_output  LeftPortType=input  RightPortType=output  PseudoPeriodic=off  Frequencies=[]  VectorFormat=inherit  Unit=inherit  AffineConversion=off
  Voltage Sensor : fl_lib/Electrical/Electrical Sensors/Voltage Sensor
  + : PMIOPort  Side=Left
  - : PMIOPort  Port=2  Side=Right
  V : Outport
  wires:
  PS-Simulink Converter/1 -> V/1
  connections:
  Voltage Sensor/RConn2 -- -/RConn1
  Voltage Sensor/LConn1 -- +/RConn1
  PS-Simulink Converter/LConn1 -- Voltage Sensor/RConn1

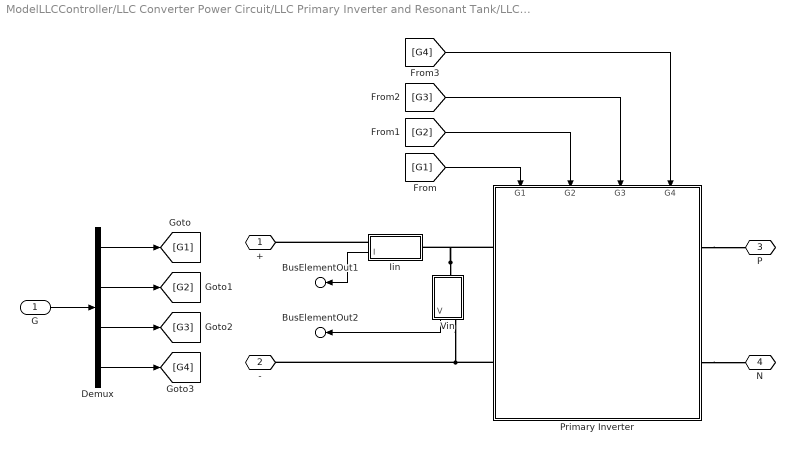
== system ModelLLCController/LLC Converter Power Circuit/LLC Primary Inverter and Resonant Tank/LLC Detailed Model/Inverter ==
  G : Inport
  Demux : Demux
  Iin : Subsystem
      settings: PortSchema="{\"entries\":[{\"content\":{\"sides\":[{\"content\":{\"connectorIds\":[\"LConn1\",\"Out1\"]},\"type\":\"ConnectorPlacement.EquallySpacedRectSide\",\"uuid\":\"e749c2ff-fd60-426f-a769-b61a7dfe80d2\"},{\"content\":{\"connectorIds\":[\"RConn1\"],\"side\":\"RIGHT\"},\"type\":\"ConnectorPlacement.EquallySpacedRectSide\",\"uuid\":\"f3bb02bd-f8d2-4326-b68c-6f969fa4ac22\"},{\"content\":{\"side\":\"TOP\"},\"type\":\"ConnectorPlacement.EquallySpacedRectSide\",\"uuid\":\"9ab7a0d1-20d8-49e4-8eb3-54d34434204c\"}]},\"type\":\"ConnectorPlacement.EquallySpacedConnector\",\"uuid\":\"19e2a6d5-13f4-47de-bb59-b826817cba83\"}],\"packageUris\":[\"http://schema.mathworks.com/mf0/Connector/R2020b\"],\"version\":\"1.0\"}"
      mask Display: disp("I")
  Primary Inverter : Subsystem  Variant=on  VariantControlMode=label  LabelModeActiveChoice=FullBridgewithoutThermal
      settings: PortSchema="{\"entries\":[{\"content\":{\"sides\":[{\"content\":{\"connectorIds\":[\"LConn1\",\"LConn2\"]},\"type\":\"ConnectorPlacement.EquallySpacedRectSide\",\"uuid\":\"27c41940-d662-4779-afdd-48b642f77411\"},{\"content\":{\"connectorIds\":[\"RConn1\",\"RConn2\"],\"side\":\"RIGHT\"},\"type\":\"ConnectorPlacement.EquallySpacedRectSide\",\"uuid\":\"b0072b01-add1-4b0f-b94e-e1b6c9886b0e\"},{\"content\":{\"connectorIds\":[\"In1\",\"In2\",\"In3\",\"In4\"],\"side\":\"TOP\"},\"type\":\"ConnectorPlacement.EquallySpacedRectSide\",\"uuid\":\"c43bed80-422d-49db-9596-8b38d5c3e411\"},{\"content\":{\"side\":\"BOTTOM\"},\"type\":\"ConnectorPlacement.EquallySpacedRectSide\",\"uuid\":\"01f06046-f57e-45b0-bca5-368a5a543f97\"}]},\"type\":\"ConnectorPlacement.EquallySpacedConnector\",\"uuid\":\"2fcb5370-6bd7-4702-bf87-ebedbb7e376c\"}],\"packageUris\":[\"http://schema.mathworks.com/mf0/Connector/R2020b\"],\"version\":\"1.0\"}"
  Vin : Subsystem
      mask Display: disp("V")
  + : PMIOPort  Side=Left
  - : PMIOPort  Port=2  Side=Left
  P : PMIOPort  Port=3  Side=Right
  N : PMIOPort  Port=4  Side=Right
  BusElementOut2 : Outport  PortName=meas  Element=VIn [V]
  BusElementOut1 : Outport  PortName=meas  Element=Iin [A]
  wires:
  Iin/1(I) -> BusElementOut1/1
  Vin/1(V) -> BusElementOut2/1
  Demux/4 -> [G4]
  Demux/3 -> [G3]
  Demux/2 -> [G2]
  Demux/1 -> [G1]
  G/1 -> Demux/1
  [G1] -> Primary Inverter/1(G1)
  [G2] -> Primary Inverter/2(G2)
  [G3] -> Primary Inverter/3(G3)
  [G4] -> Primary Inverter/4(G4)
  connections:
  Iin/LConn1 -- +/RConn1
  Vin/LConn1 -- Iin/RConn1 -- Primary Inverter/LConn1
  Vin/RConn1 -- -/RConn1 -- Primary Inverter/LConn2
  Primary Inverter/RConn1 -- P/RConn1
  Primary Inverter/RConn2 -- N/RConn1

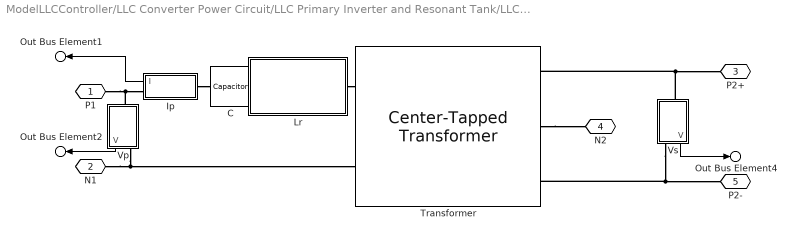
== system ModelLLCController/LLC Converter Power Circuit/LLC Primary Inverter and Resonant Tank/LLC Detailed Model/Resonant Tank ==
  C : fl_lib/Electrical/Electrical Elements/Capacitor  c=Cr F  r=0 Ohm  g=0 1/Ohm  i_specify=off  i_priority=None  i=0 A  i_nominal_specify=off  i_nominal_value=1  i_nominal_unit=A  v_specify=off  v_priority=None  v=0 V  v_nominal_specify=off  v_nominal_value=1  v_nominal_unit=V  vc_specify=off  vc_priority=None  vc=0 V  vc_nominal_specify=off  vc_nominal_value=1  vc_nominal_unit=V
  Ip : Subsystem
      settings: PortSchema="{\"entries\":[{\"content\":{\"sides\":[{\"content\":{\"connectorIds\":[\"Out1\",\"LConn1\"]},\"type\":\"ConnectorPlacement.EquallySpacedRectSide\",\"uuid\":\"e749c2ff-fd60-426f-a769-b61a7dfe80d2\"},{\"content\":{\"connectorIds\":[\"RConn1\"],\"side\":\"RIGHT\"},\"type\":\"ConnectorPlacement.EquallySpacedRectSide\",\"uuid\":\"f3bb02bd-f8d2-4326-b68c-6f969fa4ac22\"},{\"content\":{\"side\":\"TOP\"},\"type\":\"ConnectorPlacement.EquallySpacedRectSide\",\"uuid\":\"9ab7a0d1-20d8-49e4-8eb3-54d34434204c\"}]},\"type\":\"ConnectorPlacement.EquallySpacedConnector\",\"uuid\":\"19e2a6d5-13f4-47de-bb59-b826817cba83\"}],\"packageUris\":[\"http://schema.mathworks.com/mf0/Connector/R2020b\"],\"version\":\"1.0\"}"
      mask Display: disp("I")
  Lr : Subsystem  Variant=on  VariantControlMode=label  LabelModeActiveChoice=LeakageInductance
  Transformer : ee_lib/Passive/Transformers/Center-Tapped Transformer  modeling_option=ee.enum.transformer_option.nonideal  n=xfmrTurnsRatio  T=0.5  Rw1=R1 Ohm  L1=xfmrPrimaryLeakage H  Rw2=R2 Ohm  L2=xfmrSecondaryLeakage H  Rm=10000 Ohm  Lm=Lm H  i1_specify=off  i1_priority=None  i1=0 A  i1_nominal_specify=off  i1_nominal_value=1  i1_nominal_unit=A  i2p_specify=off  i2p_priority=None  i2p=0 A  i2p_nominal_specify=off  i2p_nominal_value=1  i2p_nominal_unit=A  i2n_specify=off  i2n_priority=None  i2n=0 A  i2n_nominal_specify=off  i2n_nominal_value=1  i2n_nominal_unit=A
  Vp : Subsystem
      mask Display: disp("V")
  Vs : Subsystem
      mask Display: disp("V")
  P1 : PMIOPort  Side=Left
  N1 : PMIOPort  Port=2  Side=Left
  P2+ : PMIOPort  Port=3  Side=Right
  N2 : PMIOPort  Port=4  Side=Right
  P2- : PMIOPort  Port=5  Side=Right
  Out Bus Element1 : Outport  PortName=meas  Element=Ip [A]
  Out Bus Element2 : Outport  PortName=meas  Element=Vp [V]
  Out Bus Element4 : Outport  PortName=meas  Element=Vs [A]
  wires:
  Vp/1(V) -> Out Bus Element2/1
  Ip/1(I) -> Out Bus Element1/1
  Vs/1(V) -> Out Bus Element4/1
  connections:
  Ip/RConn1 -- C/LConn1
  Vp/RConn1 -- N1/RConn1 -- Transformer/LConn2
  Vs/RConn1 -- P2-/RConn1 -- Transformer/RConn3
  Vs/LConn1 -- P2+/RConn1 -- Transformer/RConn1
  P1/RConn1 -- Vp/LConn1 -- Ip/LConn1
  Transformer/RConn2 -- N2/RConn1
  C/RConn1 -- Lr/LConn1
  Lr/RConn1 -- Transformer/LConn1

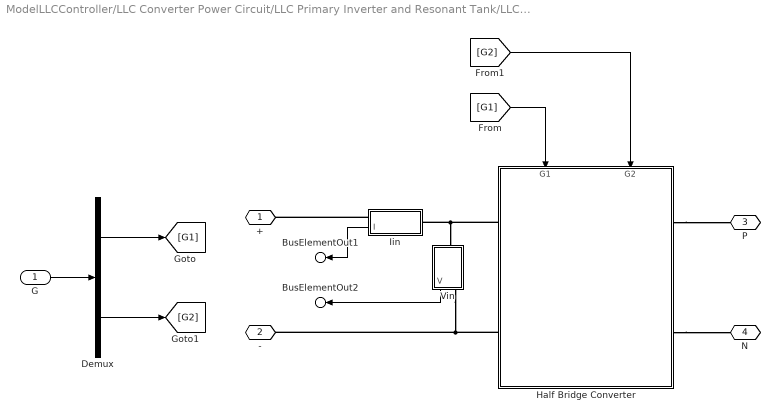
== system ModelLLCController/LLC Converter Power Circuit/LLC Primary Inverter and Resonant Tank/LLC Simplified Model/Inverter ==
  G : Inport
  Demux : Demux  Outputs=2
  Half Bridge Converter : Subsystem
      settings: PortSchema="{\"entries\":[{\"content\":{\"sides\":[{\"content\":{\"connectorIds\":[\"LConn1\",\"LConn2\"]},\"type\":\"ConnectorPlacement.EquallySpacedRectSide\",\"uuid\":\"ebe743fe-1a60-43cd-bfc1-9c2de9014673\"},{\"content\":{\"connectorIds\":[\"RConn1\",\"RConn2\"],\"side\":\"RIGHT\"},\"type\":\"ConnectorPlacement.EquallySpacedRectSide\",\"uuid\":\"437fde4e-b78c-4bc3-98e2-7afae83b9c31\"},{\"content\":{\"connectorIds\":[\"In1\",\"In2\"],\"side\":\"TOP\"},\"type\":\"ConnectorPlacement.EquallySpacedRectSide\",\"uuid\":\"02a817bf-01bb-4e65-ac43-460d77f766db\"}]},\"type\":\"ConnectorPlacement.EquallySpacedConnector\",\"uuid\":\"a9d3f8a9-dbfc-40d8-886e-239d9468324c\"}],\"packageUris\":[\"http://schema.mathworks.com/mf0/Connector/R2020b\"],\"version\":\"1.0\"}"
  Iin : Subsystem
      settings: PortSchema="{\"entries\":[{\"content\":{\"sides\":[{\"content\":{\"connectorIds\":[\"LConn1\",\"Out1\"]},\"type\":\"ConnectorPlacement.EquallySpacedRectSide\",\"uuid\":\"e749c2ff-fd60-426f-a769-b61a7dfe80d2\"},{\"content\":{\"connectorIds\":[\"RConn1\"],\"side\":\"RIGHT\"},\"type\":\"ConnectorPlacement.EquallySpacedRectSide\",\"uuid\":\"f3bb02bd-f8d2-4326-b68c-6f969fa4ac22\"},{\"content\":{\"side\":\"TOP\"},\"type\":\"ConnectorPlacement.EquallySpacedRectSide\",\"uuid\":\"9ab7a0d1-20d8-49e4-8eb3-54d34434204c\"}]},\"type\":\"ConnectorPlacement.EquallySpacedConnector\",\"uuid\":\"19e2a6d5-13f4-47de-bb59-b826817cba83\"}],\"packageUris\":[\"http://schema.mathworks.com/mf0/Connector/R2020b\"],\"version\":\"1.0\"}"
      mask Display: disp("I")
  Vin : Subsystem
      mask Display: disp("V")
  + : PMIOPort  Side=Left
  - : PMIOPort  Port=2  Side=Left
  P : PMIOPort  Port=3  Side=Right
  N : PMIOPort  Port=4  Side=Right
  BusElementOut2 : Outport  PortName=meas  Element=VIn [V]
  BusElementOut1 : Outport  PortName=meas  Element=Iin [A]
  wires:
  Iin/1(I) -> BusElementOut1/1
  Vin/1(V) -> BusElementOut2/1
  Demux/2 -> [G2]
  Demux/1 -> [G1]
  G/1 -> Demux/1
  [G1] -> Half Bridge Converter/1(G1)
  [G2] -> Half Bridge Converter/2(G2)
  connections:
  Iin/LConn1 -- +/RConn1
  Half Bridge Converter/LConn1 -- Iin/RConn1 -- Vin/LConn1
  Vin/RConn1 -- Half Bridge Converter/LConn2 -- -/RConn1
  Half Bridge Converter/RConn2 -- N/RConn1
  Half Bridge Converter/RConn1 -- P/RConn1

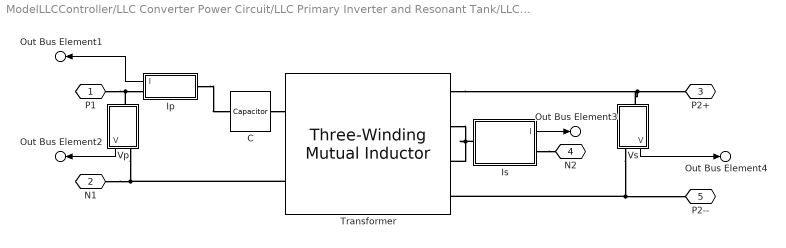
== system ModelLLCController/LLC Converter Power Circuit/LLC Primary Inverter and Resonant Tank/LLC Simplified Model/Resonant Tank ==
  C : fl_lib/Electrical/Electrical Elements/Capacitor  c=Cr F  r=0 Ohm  g=0 1/Ohm  i_specify=off  i_priority=None  i=0 A  i_nominal_specify=off  i_nominal_value=1  i_nominal_unit=A  v_specify=off  v_priority=None  v=0 V  v_nominal_specify=off  v_nominal_value=1  v_nominal_unit=V  vc_specify=off  vc_priority=None  vc=0 V  vc_nominal_specify=off  vc_nominal_value=1  vc_nominal_unit=V
  Ip : Subsystem
      settings: PortSchema="{\"entries\":[{\"content\":{\"sides\":[{\"content\":{\"connectorIds\":[\"Out1\",\"LConn1\"]},\"type\":\"ConnectorPlacement.EquallySpacedRectSide\",\"uuid\":\"e749c2ff-fd60-426f-a769-b61a7dfe80d2\"},{\"content\":{\"connectorIds\":[\"RConn1\"],\"side\":\"RIGHT\"},\"type\":\"ConnectorPlacement.EquallySpacedRectSide\",\"uuid\":\"f3bb02bd-f8d2-4326-b68c-6f969fa4ac22\"},{\"content\":{\"side\":\"TOP\"},\"type\":\"ConnectorPlacement.EquallySpacedRectSide\",\"uuid\":\"9ab7a0d1-20d8-49e4-8eb3-54d34434204c\"}]},\"type\":\"ConnectorPlacement.EquallySpacedConnector\",\"uuid\":\"19e2a6d5-13f4-47de-bb59-b826817cba83\"}],\"packageUris\":[\"http://schema.mathworks.com/mf0/Connector/R2020b\"],\"version\":\"1.0\"}"
      mask Display: disp("I")
  Is : Subsystem
      settings: PortSchema="{\"entries\":[{\"content\":{\"sides\":[{\"content\":{\"connectorIds\":[\"LConn1\",\"Out1\"]},\"type\":\"ConnectorPlacement.EquallySpacedRectSide\",\"uuid\":\"4e414c2f-0729-4c3a-890b-efd842d83184\"},{\"content\":{\"connectorIds\":[\"RConn1\"],\"side\":\"RIGHT\"},\"type\":\"ConnectorPlacement.EquallySpacedRectSide\",\"uuid\":\"a2acd69b-69fb-4c61-8702-f7ae45cb1021\"},{\"content\":{\"side\":\"TOP\"},\"type\":\"ConnectorPlacement.EquallySpacedRectSide\",\"uuid\":\"1616316f-3f63-4b85-ab48-14b40e401de5\"}]},\"type\":\"ConnectorPlacement.EquallySpacedConnector\",\"uuid\":\"70d62406-7500-443b-9d99-c073a42ed5ad\"}],\"packageUris\":[\"http://schema.mathworks.com/mf0/Connector/R2020b\"],\"version\":\"1.0\"}"
      mask Display: disp("I")
  Transformer : ee_lib/Passive/Transformers/Three-Winding Mutual Inductor  L1=Lm+Llk1 H  L2=Lm/n^2+Llk2 H  L3=Lm/n^2+Llk2 H  perfectCoupling=false  K12=Lm/sqrt((Lm+Llk1)*(Lm+n^2*Llk2))  K13=Lm/sqrt(Lm+n^2*Llk2)  K23=Lm/sqrt(Lm+n^2*Llk2)  i1_specify=off  i1_priority=None  i1=0 A  i1_nominal_specify=off  i1_nominal_value=1  i1_nominal_unit=A  i2_specify=off  i2_priority=None  i2=0 A  i2_nominal_specify=off  i2_nominal_value=1  i2_nominal_unit=A  i3_specify=off  i3_priority=None  i3=0 A  i3_nominal_specify=off  i3_nominal_value=1  i3_nominal_unit=A
  Vp : Subsystem
      mask Display: disp("V")
  Vs : Subsystem
      mask Display: disp("V")
  P1 : PMIOPort  Side=Left
  N1 : PMIOPort  Port=2  Side=Left
  P2+ : PMIOPort  Port=3  Side=Right
  N2 : PMIOPort  Port=4  Side=Right
  P2-- : PMIOPort  Port=5  Side=Right
  Out Bus Element1 : Outport  PortName=meas  Element=Ip [A]
  Out Bus Element2 : Outport  PortName=meas  Element=Vp [V]
  Out Bus Element3 : Outport  PortName=meas  Element=Is [A]
  Out Bus Element4 : Outport  PortName=meas  Element=Vs [A]
  wires:
  Vp/1(V) -> Out Bus Element2/1
  Ip/1(I) -> Out Bus Element1/1
  Vs/1(V) -> Out Bus Element4/1
  Is/1(I) -> Out Bus Element3/1
  connections:
  C/RConn1 -- Transformer/LConn1
  Ip/RConn1 -- C/LConn1
  Vp/RConn1 -- Transformer/LConn2 -- N1/RConn1
  Vs/RConn1 -- Transformer/RConn4 -- P2--/RConn1
  Vs/LConn1 -- Transformer/RConn1 -- P2+/RConn1
  P1/RConn1 -- Vp/LConn1 -- Ip/LConn1
  Transformer/RConn2 -- Is/RConn1 -- Transformer/RConn3
  Is/LConn1 -- N2/RConn1
